simulink model "reachout_visual_rotation"  (Simulink 8.1)
settings: Solver=ode4  SolverMode=SingleTasking  StartTime=0.0  StopTime=inf  FixedStep=0.0005  RelTol=1e-3
model workspace (MAT data in the model file):
  BKIN_STEP_TIME = 0.0005
  col_x = 1
  col_y = 2
  E_TARGET_ON = 3
  E_HOLD_AT_TARGET = 5
  LOGICAL_RADIUS = 4
  START_TARGET_COL = 1
  END_TARGET_COL = 2
  ROTATION_CENTER = 3
  WAIT_AT_1stTARGET_COL = 4
  MAXREACHTIME_COL = 5
  WAIT_AT_2ndTARGET_COL = 6
  ROTATION_TYPE = 8
  ROTATION = 9
  DELAY_POSTTRIAL_COL = 7
  E_STAY_CENTER = 2
  VISUAL_RADIUS = 3
  COLOR = 5
  ALTCOLOR : num (value not decoded)
StartFcn:
  |  warndlg('Dexterit-E models cannot run under simulation. Please compile your model and run it from within Dexterit-E.');set_param(bdroot,'SimulationCommand','stop')
undefined symbols (not defined in the file or in its folder): slselsubs
libraries: General x3, Video x3, KINARM_general x1
CloseFcn:
  | rtwprivate ssgencode ModelCloseRequest b2lab2d
settings Model: Creator=Chris Grebeldinger  LastModifiedBy=dmclean  ModifiedComment=chris -- Wed Feb 16 09:18:30 2005 -- Version 1.1384  ModifiedHistory=Feb 16/05 - Add error repeat, add offset ramp  ExtModeArmWhenConnect=off  ExtModeLogAll=off  BufferReuse=off
settings DataIOCC: LimitDataPoints=off  SaveOutput=off  SaveTime=off  SignalLoggingName=sigsOut
settings OptimizationCC: BlockReduction=off  BooleanDataType=off  OptimizeBlockIOStorage=off  BufferReuse=off  ExpressionFolding=off  FoldNonRolledExpr=off  LocalBlockOutputs=off  InitFltsAndDblsToZero=on
settings DebuggingCC: SaveWithParameterizedLinksMsg=none  SignalResolutionControl=TryResolveAllWithWarning  SolverPrmCheckMsg=none  MultiTaskDSMMsg=warning  MultiTaskCondExecSysMsg=none  StrictBusMsg=None
settings HardwareCC: ProdIntDivRoundTo=Zero  ProdEndianess=LittleEndian  ProdHWDeviceType=Generic->32-bit x86 compatible  TargetHWDeviceType=32-bit Generic
settings SFSimCC: SimParseCustomCode=off
settings RTWCC: SystemTargetFile=xpctarget.tlc  TemplateMakefile=xpc_default_tmf  Description=xPC Target  ProcessScript=xpctarget_make_rtw_hook  IncludeERTFirstTime=on  RTWCompilerOptimization=On
settings CodeAppCC: MaxIdLength=63
settings xpcTargetCC: TargetFcnLib=ansi_tfl_tmw.mat  CodeReplacementLibrary=XPC_BLAS  ParMdlRefBuildCompliant=on  ConcurrentExecutionCompliant=on  CombineSignalStateStructs=off  MATLABClassNameForMDSCustomization=xpcAperiodicCustomization  GRTInterface=on  GenerateAllocFcn=off  xPCTaskExecutionProfile=off  xPCRL32EventNumber=5000  xPCisDownloadable=off  xPCLoadParamSetFile=off  xPCConcurrentTasks=off  xPCEnableSFAnimation=off

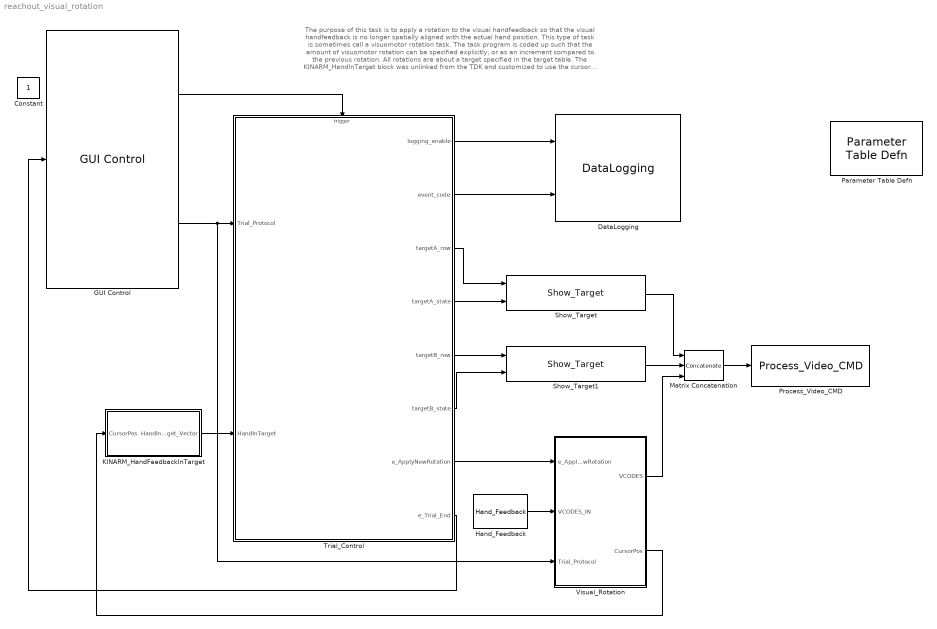
== system reachout_visual_rotation ==
  note: The purpose of this task is to apply a rotation to the visual handfeedback so that the visual handfeedback is no longer spatially aligned with the actual hand position.
      | This type of task is sometimes call a visuomotor rotation task.
      | The task program is coded up such that the amount of visuomotor rotation can be specified explicitly, or as an increment compared to the previous rotation.
      | All rotations are about a target specified in the target table.
      |
      | The KINARM_HandInTarget block was unlinked from the TDK and customized to use the cursor position as hand feedback input, rather than the KINARM robot's actual location.
  DataLogging : General/DataLogging  log_event_codes=on  log_analog_inputs=off
  GUI Control : General/GUI Control  target_type_str=Circle  Target_Type=1  XYcols=[1 2]  Vcols=3  Lcols=4  indices_padding=[0 0 0 0;0 0 0 0]  task_version=1.0  show_repeat_trial_flag=off
  Hand_Feedback : KINARM_general/Hand_Feedback  feedback_cntl_src=none
  KINARM_HandFeedbackInTarget : Subsystem  AncestorBlock=KINARM_general/KINARM_HandInTarget  mask(KINARM_HandInTarget){use_dominant_hand=on, target_type=Circle, num_states=1, attribcol1=4, attribcol2=3, attribcol3=3, attribcol4=3}
      mask prompts: use_dominant_hand "Dominant Hand?"; target_type "Type of Target"; num_states "Number of Target States"; attribcol1 "State 1 Target Table Column(s)"; attribcol2 "State 2 Target Table Column(s)"; attribcol3 "State 3 Target Table Column(s)"; attribcol4 "State 4 Target Table Column(s)"
      mask help: This block returns a vector or array corresponding to the Target_Table rows indicating whether the specified hand is in (=1) or out (=0) of each of the targets.
      mask init:
      | num_states=str2num(get_param(gcb, 'num_states'));
      | columntext='(columns: ';
      | 
      | for i=1:num_states
      | 	varname=['attribcol' num2str(i)];
      | 	if i>1
      | 		columntext=[columntext, '; '];
      | 	end
      | 	columntext=[columntext, get_param(gcb, varname)];
      | end
      | columntext=strvcat([columntext ')'],' ', ' ');
      | 
      | output_block=char(find_system(gcb,'LookUnderMasks','all','FollowLinks','on','SearchDepth',1,'BlockType','Outport'));
      | outputname=get_param(output_block,'Name');
      | 
      | % Select only the desired states for output. The output port is also renamed to reflect 
      | % whether the output is a vector (in the case of a single state) or an array (of vectors, 
      | % one for each of multiple states).
      | if num_states == 1
      | 	set_param([gcb '/Selected States'], 'Value', '[1]');
      | 	set_param(output_block, 'Name', 'HandInTarget_Vector');
      | elseif num_states == 2
      | 	set_param([gcb '/Selected States'], 'Value', '[1,2]');
      | 	set_param(output_block, 'Name', 'HandInTarget_Array');
      | elseif num_states == 3
      | 	set_param([gcb '/Selected States'], 'Value', '[1,2,3]');
      | 	set_param(output_block, 'Name', 'HandInTarget_Array');
      | else
      | 	set_param([gcb '/Selected States'], 'Value', '[1,2,3,4]');
      | 	set_param(output_block, 'Name', 'HandInTarget_Array');
      | end
      mask Help:
      | Used to determine if the hand (finger-tip) is in any of the targets in the Target_Table.
      | <P>
      | <B><I>Use of this block requires that the DataLogging block (General library) be set to log KINARM data.</I></B>
      | 
      | <H2>Library </H2>
      | KINARM_general (sub-library)
      | 
      | <H2>Description </H2>
      | This block returns a vector or array corresponding to the Target_Table rows indicating whether the specified hand (i.e. finger-tip) is in or out of each of the targets.  Each element in the output vector or output array will be either a 0 (hand not in target) or a 1 (hand in target).
      | <P>
      | A vector is returned if only one target state is specified in each target row (see Parameters and Dialog Box), with each index of the vector corresponding to a row in the target table.  An array is returned if more than one target state is specified in a target row, with each row of the array corresponding to a target row and each column corresponding to the nth target state specified in each target row.
      | <P>
      | The output vector or array is typically used by a stateflow chart to affect behavior of the system.  Because this block returns hand-in-target information for all targets in the target table, multiple targets can be monitored at once (i.e. the stateflow chart could have certain transitions that occur if the hand is in one target and other transitions if it is in a different target).  Likewise, because this block returns hand-in-target information for multiple states of a single target, those multiple states can be monitored simultaneously.
      | <P>
      | Because the KINARM_HandInTarget block returns information for only one hand, two copies of this block are required if information for both hands is desired.
      | <P>
      | 
      | <H2>Parameters and Dialog Box</H2>
      | <B>Dominant Hand?:</B> this box determines which hand is used by this block : dominant hand position (checked box) or the non-dominant hand position (unchecked box).  (Note: if the end-user wants to know about both the dominant hand and the non-dominant hand, then 2 separate copies of this block are requried, one for each hand.)
      | <P>
      | <B>Type of Target:</B> Enter the type of target specified in the target table:
      | <P>
      | <B>Number of Target States:</B> Enter the number of target states specified in each target row.  Up to four target states are allowed per target row.
      | <P>
      | <B>State <n> Target Table Columns:</B> Enter the columns in the Target Table that specify the relevant target attributes.  Do this for each target state.
      | For a circle, enter the columns corresponding to logical radius (e.g. 4)
      | <BR>For an ellipse, enter the columns corresponding to major radius, minor radius, rotation angle (e.g. [4, 5, 6]).
      | <BR>For a rectangle, enter the columns corresponding to length, height, and rotation angle (e.g. [4, 5, 6]).
      | <BR>For a line, enter the columns corresponding to stroke width, endpoint in x, and endpoint in y (e.g. [3, 4, 5]).
      | <BR>For a triangle, enter the columns corresponding to length, height, peak offset, and rotation angle (e.g. [4, 5, 6, 7]).
      | 
      | <H2>Examples</H2>
      | <B>Example 1.</B>  Suppose a target row will be used to define 1 state for a circle type target and the radius of the visual target is the same radius to be used for determination of hand-in-target.  The related Target Table column is: column 6 = radius.  For this example, "State 1 Target Table Columns" would equal [6].
      | <P>
      | 
      | <B>Example 2.</B>  Suppose a target row will be used to define 1 state for a circle type target, but the radius of the visual target will be different than the radius to be used for determination of hand-in-target.  This option allows independent control over the size of the visual target versus the accuracy needed to be considered "in the target".  The related Target Table columns are: column 6 = radius1 (i.e. radius to target to be drawn); column 7 = radius2 (i.e. radius to be used for hand-in-target) .  For this example, "State 1 Target Table Columns" would equal [7].
      | <P>
      | <B>Example 3.</B>  Suppose a target row will be used to define 2 states for a circle type target, where the radius of the visual target will be a constant, but depending on the state of the system, one of 2 other and different radii will be used for determination of hand-in-target.  The related Target Table columns are: column 6 = radius1 (i.e. radius to target to be drawn); column 7 = radius2 (i.e. radius to be used for hand-in-target for state 1); column 8 = radius3 (i.e. radius to be used for hand-in-target for state 2).  For this example, "State 1 Target Table Columns" would equal [7], while "State 2 Target Table Columns" would equal [8].
      | <P>
      | 
      | <H2>Related Blocks </H2>
      | DataLogging
      mask TypeOptions target_type: Circle | Ellipse | Rectangle | Line | Triangle
      mask Callback target_type:
      | target_type=get_param(gcb, 'target_type');
      | attribcol1=[str2num(get_param(gcb, 'attribcol1')) 0 0 0 0 0 0];
      | attribcol2=[str2num(get_param(gcb, 'attribcol2')) 0 0 0 0 0 0];
      | attribcol3=[str2num(get_param(gcb, 'attribcol3')) 0 0 0 0 0 0];
      | attribcol4=[str2num(get_param(gcb, 'attribcol4')) 0 0 0 0 0 0];
      | switch target_type(1:3)
      | 	case 'Cir'
      | 		numcol=1;
      | 	case 'Ell'
      | 		numcol=3;
      |     case 'Rec'
      |         numcol=3;
      |     case 'Lin'
      |         numcol=3;
      |     case 'Tri'
      |         numcol=4;
      | 	otherwise
      | 		numcol=1;
      | end
      | if numcol==1
      | 	set_param(gcb, 'attribcol1', num2str(attribcol1(1)));
      | 	set_param(gcb, 'attribcol2', num2str(attribcol2(1)));
      | 	set_param(gcb, 'attribcol3', num2str(attribcol3(1)));
      | 	set_param(gcb, 'attribcol4', num2str(attribcol4(1)));
      | else
      | 	set_param(gcb, 'attribcol1', ['[' num2str(attribcol1(1:numcol)) ']']);
      | 	set_param(gcb, 'attribcol2', ['[' num2str(attribcol2(1:numcol)) ']']);
      | 	set_param(gcb, 'attribcol3', ['[' num2str(attribcol3(1:numcol)) ']']);
      | 	set_param(gcb, 'attribcol4', ['[' num2str(attribcol4(1:numcol)) ']']);
      | end
      mask TypeOptions num_states: 1 | 2 | 3 | 4
      mask Callback num_states:
      | num_states = str2num(get_param(gcb, 'num_states'));
      | vis = get_param(gcb, 'MaskVisibilities');
      | 
      | % Select only the desired states for output. The output port is also renamed to reflect
      | % whether the output is a vector (in the case of a single state) or an array (of vectors,
      | % one for each of multiple states).
      | output_block=char(find_system(gcb, 'LookUnderMasks', 'all', 'FollowLinks', 'on', 'SearchDepth', 1, 'BlockType', 'Outport'));
      | 
      | if num_states == 1
      | 	set_param([gcb '/Selected States'], 'Value', '[1]');
      | 	set_param(output_block, 'Name', 'HandInTarget_Vector');
      | 	vis{5} = 'off';
      | 	vis{6} = 'off';
      | 	vis{7} = 'off';
      | elseif num_states == 2
      | 	set_param([gcb '/Selected States'], 'Value', '[1,2]');
      | 	set_param(output_block, 'Name', 'HandInTarget_Array');
      | 	vis{5} = 'on';
      | 	vis{6} = 'off';
      | 	vis{7} = 'off';
      | elseif num_states == 3
      | 	set_param([gcb '/Selected States'], 'Value', '[1,2,3]');
      | 	set_param(output_block, 'Name','HandInTarget_Array');
      | 	vis{5} = 'on';
      | 	vis{6} = 'on';
      | 	vis{7} = 'off';
      | else
      | 	set_param([gcb '/Selected States'], 'Value', '[1,2,3,4]');
      | 	set_param(output_block, 'Name', 'HandInTarget_Array');
      | 	vis{5} = 'on';
      | 	vis{6} = 'on';
      | 	vis{7} = 'on';
      | end
      | set_param(gcb, 'MaskVisibilities', vis);
      | 
      | target_type=get_param(gcb, 'target_type');
      | attribcol1=[str2num(get_param(gcb, 'attribcol1')) 0 0 0 0 0 0];
      | attribcol2=[str2num(get_param(gcb, 'attribcol2')) 0 0 0 0 0 0];
      | attribcol3=[str2num(get_param(gcb, 'attribcol3')) 0 0 0 0 0 0];
      | attribcol4=[str2num(get_param(gcb, 'attribcol4')) 0 0 0 0 0 0];
      | switch target_type(1:3)
      | 	case 'Cir'
      | 		numcol=1;
      | 	case 'Ell'
      | 		numcol=3;
      |     case 'Rec'
      |         numcol=3;
      |     case 'Lin'
      |         numcol=3;
      |     case 'Tri'
      |         numcol=4;
      | 	otherwise
      | 		numcol=1;
      | end
      | if numcol==1
      | 	set_param(gcb, 'attribcol1', num2str(attribcol1(1)));
      | 	set_param(gcb, 'attribcol2', num2str(attribcol2(1)));
      | 	set_param(gcb, 'attribcol3', num2str(attribcol3(1)));
      | 	set_param(gcb, 'attribcol4', num2str(attribcol4(1)));
      | else
      | 	set_param(gcb, 'attribcol1', ['[' num2str(attribcol1(1:numcol)) ']']);
      | 	set_param(gcb, 'attribcol2', ['[' num2str(attribcol2(1:numcol)) ']']);
      | 	set_param(gcb, 'attribcol3', ['[' num2str(attribcol3(1:numcol)) ']']);
      | 	set_param(gcb, 'attribcol4', ['[' num2str(attribcol4(1:numcol)) ']']);
      | end
      mask Callback attribcol1:
      | target_type=get_param(gcb, 'target_type');
      | attribcol1=[str2num(get_param(gcb, 'attribcol1')) 0 0 0 0 0 0];
      | attribcol2=[str2num(get_param(gcb, 'attribcol2')) 0 0 0 0 0 0];
      | attribcol3=[str2num(get_param(gcb, 'attribcol3')) 0 0 0 0 0 0];
      | attribcol4=[str2num(get_param(gcb, 'attribcol4')) 0 0 0 0 0 0];
      | switch target_type(1:3)
      | 	case 'Cir'
      | 		numcol=1;
      | 	case 'Ell'
      | 		numcol=3;
      |     case 'Rec'
      |         numcol=3;
      |     case 'Lin'
      |         numcol=3;
      |     case 'Tri'
      |         numcol=4;
      | 	otherwise
      | 		numcol=1;
      | end
      | if numcol==1
      | 	set_param(gcb, 'attribcol1', num2str(attribcol1(1)));
      | 	set_param(gcb, 'attribcol2', num2str(attribcol2(1)));
      | 	set_param(gcb, 'attribcol3', num2str(attribcol3(1)));
      | 	set_param(gcb, 'attribcol4', num2str(attribcol4(1)));
      | else
      | 	set_param(gcb, 'attribcol1', ['[' num2str(attribcol1(1:numcol)) ']']);
      | 	set_param(gcb, 'attribcol2', ['[' num2str(attribcol2(1:numcol)) ']']);
      | 	set_param(gcb, 'attribcol3', ['[' num2str(attribcol3(1:numcol)) ']']);
      | 	set_param(gcb, 'attribcol4', ['[' num2str(attribcol4(1:numcol)) ']']);
      | end
      mask Callback attribcol2:
      | target_type=get_param(gcb, 'target_type');
      | attribcol1=[str2num(get_param(gcb, 'attribcol1')) 0 0 0 0 0 0];
      | attribcol2=[str2num(get_param(gcb, 'attribcol2')) 0 0 0 0 0 0];
      | attribcol3=[str2num(get_param(gcb, 'attribcol3')) 0 0 0 0 0 0];
      | attribcol4=[str2num(get_param(gcb, 'attribcol4')) 0 0 0 0 0 0];
      | switch target_type(1:3)
      | 	case 'Cir'
      | 		numcol=1;
      | 	case 'Ell'
      | 		numcol=3;
      |     case 'Rec'
      |         numcol=3;
      |     case 'Lin'
      |         numcol=3;
      |     case 'Tri'
      |         numcol=4;
      | 	otherwise
      | 		numcol=1;
      | end
      | if numcol==1
      | 	set_param(gcb, 'attribcol1', num2str(attribcol1(1)));
      | 	set_param(gcb, 'attribcol2', num2str(attribcol2(1)));
      | 	set_param(gcb, 'attribcol3', num2str(attribcol3(1)));
      | 	set_param(gcb, 'attribcol4', num2str(attribcol4(1)));
      | else
      | 	set_param(gcb, 'attribcol1', ['[' num2str(attribcol1(1:numcol)) ']']);
      | 	set_param(gcb, 'attribcol2', ['[' num2str(attribcol2(1:numcol)) ']']);
      | 	set_param(gcb, 'attribcol3', ['[' num2str(attribcol3(1:numcol)) ']']);
      | 	set_param(gcb, 'attribcol4', ['[' num2str(attribcol4(1:numcol)) ']']);
      | end
      mask Callback attribcol3:
      | target_type=get_param(gcb, 'target_type');
      | attribcol1=[str2num(get_param(gcb, 'attribcol1')) 0 0 0 0 0 0];
      | attribcol2=[str2num(get_param(gcb, 'attribcol2')) 0 0 0 0 0 0];
      | attribcol3=[str2num(get_param(gcb, 'attribcol3')) 0 0 0 0 0 0];
      | attribcol4=[str2num(get_param(gcb, 'attribcol4')) 0 0 0 0 0 0];
      | switch target_type(1:3)
      | 	case 'Cir'
      | 		numcol=1;
      | 	case 'Ell'
      | 		numcol=3;
      |     case 'Rec'
      |         numcol=3;
      |     case 'Lin'
      |         numcol=3;
      |     case 'Tri'
      |         numcol=4;
      | 	otherwise
      | 		numcol=1;
      | end
      | if numcol==1
      | 	set_param(gcb, 'attribcol1', num2str(attribcol1(1)));
      | 	set_param(gcb, 'attribcol2', num2str(attribcol2(1)));
      | 	set_param(gcb, 'attribcol3', num2str(attribcol3(1)));
      | 	set_param(gcb, 'attribcol4', num2str(attribcol4(1)));
      | else
      | 	set_param(gcb, 'attribcol1', ['[' num2str(attribcol1(1:numcol)) ']']);
      | 	set_param(gcb, 'attribcol2', ['[' num2str(attribcol2(1:numcol)) ']']);
      | 	set_param(gcb, 'attribcol3', ['[' num2str(attribcol3(1:numcol)) ']']);
      | 	set_param(gcb, 'attribcol4', ['[' num2str(attribcol4(1:numcol)) ']']);
      | end
      mask Callback attribcol4:
      | target_type=get_param(gcb, 'target_type');
      | attribcol1=[str2num(get_param(gcb, 'attribcol1')) 0 0 0 0 0 0];
      | attribcol2=[str2num(get_param(gcb, 'attribcol2')) 0 0 0 0 0 0];
      | attribcol3=[str2num(get_param(gcb, 'attribcol3')) 0 0 0 0 0 0];
      | attribcol4=[str2num(get_param(gcb, 'attribcol4')) 0 0 0 0 0 0];
      | switch target_type(1:3)
      | 	case 'Cir'
      | 		numcol=1;
      | 	case 'Ell'
      | 		numcol=3;
      |     case 'Rec'
      |         numcol=3;
      |     case 'Lin'
      |         numcol=3;
      |     case 'Tri'
      |         numcol=4;
      | 	otherwise
      | 		numcol=1;
      | end
      | if numcol==1
      | 	set_param(gcb, 'attribcol1', num2str(attribcol1(1)));
      | 	set_param(gcb, 'attribcol2', num2str(attribcol2(1)));
      | 	set_param(gcb, 'attribcol3', num2str(attribcol3(1)));
      | 	set_param(gcb, 'attribcol4', num2str(attribcol4(1)));
      | else
      | 	set_param(gcb, 'attribcol1', ['[' num2str(attribcol1(1:numcol)) ']']);
      | 	set_param(gcb, 'attribcol2', ['[' num2str(attribcol2(1:numcol)) ']']);
      | 	set_param(gcb, 'attribcol3', ['[' num2str(attribcol3(1:numcol)) ']']);
      | 	set_param(gcb, 'attribcol4', ['[' num2str(attribcol4(1:numcol)) ']']);
      | end
      mask Display:
      | disp(columntext)
      | port_label('output',1,outputname)
  Matrix Concatenation : Concatenate  NumInputs=3  Mode=Multidimensional array
  Parameter Table Defn : General/Parameter Table Defn  ShowInLibBrowser=0
  Process_Video_CMD : Video/Process_Video_CMD
  Show_Target : Video/Show_Target  target_type=Circle  num_states=2  attribcol1=[COLOR 0 0 VISUAL_RADIUS]  attribcol2=[ALTCOLOR 0 0 VISUAL_RADIUS]  attribcol3=[0 0 0 0]  attribcol4=[0 0 0 0]  attribcol5=[0 0 24 0]  stateindices_padding=[0 0 0 0 0 0 0;0 0 0 0 0 0 0;0 0 0 0 0 0 0;0 0 0 0 0 0 0;0 0 0 0 0 0 0]  source=dialog  opacity=100  target_display=Both subject and operator displays  num_col=4
  Show_Target1 : Video/Show_Target  target_type=Circle  num_states=2  attribcol1=[COLOR 0 0 VISUAL_RADIUS]  attribcol2=[ALTCOLOR 0 0 VISUAL_RADIUS]  attribcol3=[0 0 0 0]  attribcol4=[0 0 0 0]  attribcol5=[0 0 24 0]  stateindices_padding=[0 0 0 0 0 0 0;0 0 0 0 0 0 0;0 0 0 0 0 0 0;0 0 0 0 0 0 0;0 0 0 0 0 0 0]  source=dialog  opacity=100  target_display=Both subject and operator displays  num_col=4
  Trial_Control : Stateflow chart  TreatAsAtomicUnit=on
  Visual_Rotation : Subsystem
  Constant : Constant  IOType=siggen
  wires:
  Show_Target/1 -> Matrix Concatenation/1
  GUI Control/2 -> Trial_Control/1(Trial_Protocol), Visual_Rotation/3(Trial_Protocol)
  Trial_Control/8(e_Trial_End) -> GUI Control/1
  GUI Control/1 -> Trial_Control/Trigger
  Trial_Control/4(targetA_state) -> Show_Target/2
  Trial_Control/3(targetA_row) -> Show_Target/1
  Show_Target1/1 -> Matrix Concatenation/2
  Trial_Control/5(targetB_row) -> Show_Target1/1
  Trial_Control/6(targetB_state) -> Show_Target1/2
  Trial_Control/2(event_code) -> DataLogging/2
  Matrix Concatenation/1 -> Process_Video_CMD/1
  Hand_Feedback/1 -> Visual_Rotation/2(VCODES_IN)
  Visual_Rotation/2(CursorPos) -> KINARM_HandFeedbackInTarget/1(CursorPos)
  KINARM_HandFeedbackInTarget/1(HandInTarget_Vector) -> Trial_Control/2(HandInTarget)
  Trial_Control/7(e_ApplyNewRotation) -> Visual_Rotation/1(e_ApplyNewRotation)
  Visual_Rotation/1(VCODES) -> Matrix Concatenation/3
  Trial_Control/1(logging_enable) -> DataLogging/1

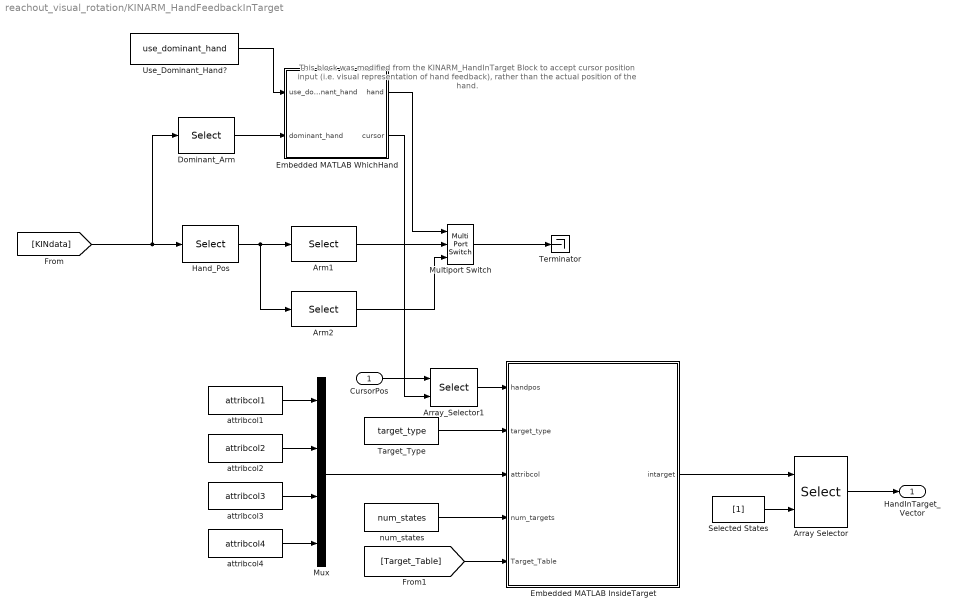
== system reachout_visual_rotation/KINARM_HandFeedbackInTarget ==
  note: This block was modified from the KINARM_HandInTarget Block to accept cursor position input (i.e. visual
      | representation of hand feedback), rather than the actual position of the hand.
  CursorPos : Inport
  Arm1 : Selector  NumberOfDimensions=2  InputPortWidth=3  IndexOptions=Index vector (dialog),Select all  Indices=1,-1  OutputSizes=slselsubs([(-2),(-2)],1),slselsubs([(-2),(-2)],2)
  Arm2 : Selector  NumberOfDimensions=2  InputPortWidth=3  IndexOptions=Index vector (dialog),Select all  Indices=2,-1  OutputSizes=slselsubs([(-2),(-2)],1),slselsubs([(-2),(-2)],2)
  Array Selector : Selector  NumberOfDimensions=2  InputPortWidth=3  IndexOptions=Select all,Index vector (port)  Indices=-1,1  OutputSizes=slselsubs([(-2),(-2)],1),slselsubs([(-2),(-2)],2)
  Array_Selector1 : Selector  NumberOfDimensions=2  InputPortWidth=3  IndexOptions=Index vector (port),Select all  Indices=-1,1  OutputSizes=1
  Dominant_Arm : Selector  NumberOfDimensions=2  InputPortWidth=3  IndexOptions=Index vector (dialog),Index vector (dialog)  Indices=[3],[1]  OutputSizes=slselsubs([(-2),(-2)],1),slselsubs([(-2),(-2)],2)
  Embedded MATLAB InsideTarget : MATLAB Function  TreatAsAtomicUnit=on
  Embedded MATLAB WhichHand : MATLAB Function  TreatAsAtomicUnit=on
  Hand_Pos : Selector  NumberOfDimensions=2  InputPortWidth=3  IndexOptions=Select all,Index vector (dialog)  Indices=-1,[23,24]  OutputSizes=slselsubs([(-2),(-2)],1),slselsubs([(-2),(-2)],2)
  Multiport Switch : MultiPortSwitch  Inputs=2
  Mux : Mux
  Selected States : Constant  Value=[1]
  Target_Type : Constant  Value=target_type
  Terminator : Terminator
  Use_Dominant_Hand? : Constant  Value=use_dominant_hand
  attribcol1 : Constant  Value=attribcol1
  attribcol2 : Constant  Value=attribcol2
  attribcol3 : Constant  Value=attribcol3
  attribcol4 : Constant  Value=attribcol4
  num_states : Constant  Value=num_states
  HandInTarget_Vector : Outport
  wires:
  Selected States/1 -> Array Selector/2
  num_states/1 -> Embedded MATLAB InsideTarget/4(num_targets)
  Mux/1 -> Embedded MATLAB InsideTarget/3(attribcol)
  attribcol4/1 -> Mux/4
  attribcol3/1 -> Mux/3
  attribcol2/1 -> Mux/2
  attribcol1/1 -> Mux/1
  Use_Dominant_Hand?/1 -> Embedded MATLAB WhichHand/1(use_dominant_hand)
  Embedded MATLAB WhichHand/1(hand) -> Multiport Switch/1
  Target_Type/1 -> Embedded MATLAB InsideTarget/2(target_type)
  Array Selector/1 -> HandInTarget_Vector/1
  [Target_Table] -> Embedded MATLAB InsideTarget/5(Target_Table)
  Embedded MATLAB InsideTarget/1(intarget) -> Array Selector/1
  Multiport Switch/1 -> Terminator/1
  Arm2/1 -> Multiport Switch/3
  Arm1/1 -> Multiport Switch/2
  Dominant_Arm/1 -> Embedded MATLAB WhichHand/2(dominant_hand)
  Hand_Pos/1 -> Arm2/1, Arm1/1
  [KINdata] -> Dominant_Arm/1, Hand_Pos/1
  CursorPos/1 -> Array_Selector1/1
  Array_Selector1/1 -> Embedded MATLAB InsideTarget/1(handpos)
  Embedded MATLAB WhichHand/2(cursor) -> Array_Selector1/2

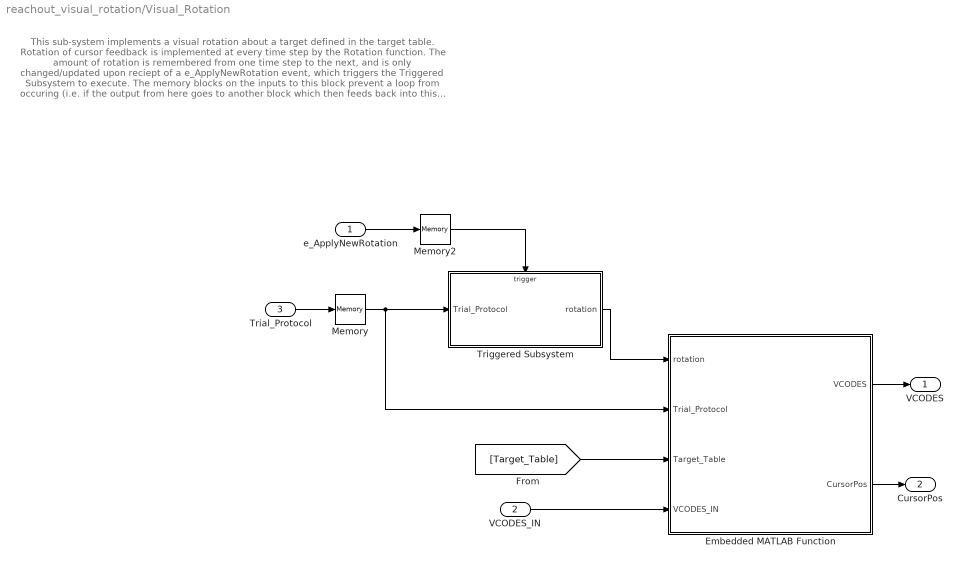
== system reachout_visual_rotation/Visual_Rotation ==
  note: This sub-system implements a visual rotation about a target defined in the target table.
      |
      | Rotation of cursor feedback is implemented at every time step by the Rotation function.
      | The amount of rotation is remembered from one time step to the next, and is only changed/updated
      | upon reciept of a e_ApplyNewRotation event, which triggers the Triggered Subsystem to execute.
      |
      | The memory blocks on the inputs to this block prevent a loop from occuring (i.e. if the output from here goes to
      | another block which then feeds back into this block, which forms a loop, which needs to be broken by the Memory block).
  e_ApplyNewRotation : Inport
  VCODES_IN : Inport  Port=2
  Trial_Protocol : Inport  Port=3
  Embedded MATLAB Function : MATLAB Function  TreatAsAtomicUnit=on
  Memory : Memory  InheritSampleTime=on
  Memory2 : Memory  InheritSampleTime=on
  Triggered Subsystem : Subsystem  TreatAsAtomicUnit=on
  VCODES : Outport
  CursorPos : Outport  Port=2
  wires:
  Trial_Protocol/1 -> Memory/1
  Embedded MATLAB Function/1(VCODES) -> VCODES/1
  VCODES_IN/1 -> Embedded MATLAB Function/4(VCODES_IN)
  Embedded MATLAB Function/2(CursorPos) -> CursorPos/1
  Memory/1 -> Triggered Subsystem/1(Trial_Protocol), Embedded MATLAB Function/2(Trial_Protocol)
  e_ApplyNewRotation/1 -> Memory2/1
  Triggered Subsystem/1(rotation) -> Embedded MATLAB Function/1(rotation)
  [Target_Table] -> Embedded MATLAB Function/3(Target_Table)
  Memory2/1 -> Triggered Subsystem/Trigger

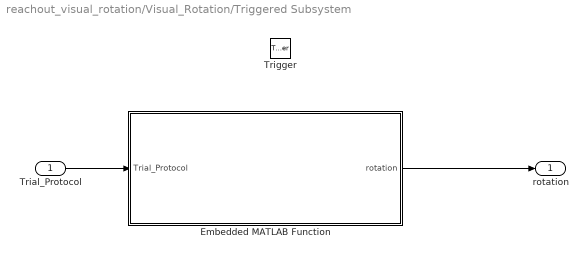
== system reachout_visual_rotation/Visual_Rotation/Triggered Subsystem ==
  Trial_Protocol : Inport
  Trigger : TriggerPort  TriggerType=either
  Embedded MATLAB Function : MATLAB Function  TreatAsAtomicUnit=on
  rotation : Outport
  wires:
  Trial_Protocol/1 -> Embedded MATLAB Function/1(Trial_Protocol)
  Embedded MATLAB Function/1(rotation) -> rotation/1

== stateflow chart Trial_Control ==
  settings: sampleTime=0.001
  state Inter_Trial_State/
    // send e_Trial_End event
    e_Trial_End;
    // turn off both targets
    // stop data logging
    event_code=0;
    targetA_state=0;
    targetB_state=0;
    logging_enable = 0;
  state Initialize/
    // Turn off both targets, set hand_feedback on
    targetA_state=0;
    targetB_state=0;
  state Main_Trial
    state Show2ndTarget/
      // Turn on second target, log an event, wait until hand-is-in-target or wait for specified delay
      event_code=E_TARGET_ON;
      targetB_row = Trial_Protocol[END_TARGET_COL];
      targetB_state=1;
      tickCount =Trial_Protocol[MAXREACHTIME_COL];
    state StayAt2ndTarget/
      // change the 2nd target's state, log an event, wait for a specified period of time
      event_code=E_HOLD_AT_TARGET;
      targetB_state=2;
      tickCount =Trial_Protocol[WAIT_AT_2ndTARGET_COL];
    state EndOfTrial/
      // Wait for a specified period of time,
      tickCount =Trial_Protocol[DELAY_POSTTRIAL_COL];
    state StayAtFirstTarget/
      // change the first target state (e.g. colour), log an event, wait for specified period of time.  Hand must STAY in target for specified time.
      logging_enable = 1;
      event_code=E_STAY_CENTER;
      targetA_state=2;
      tickCount =Trial_Protocol[WAIT_AT_1stTARGET_COL];
    state FirstTargetOn/
      // Turn on first target, set loading conditions, enable data logging, wait for specified delay or until hand-is-in-target
      targetA_row = Trial_Protocol[START_TARGET_COL];
      targetA_state=1;
    FirstTargetOn -> StayAtFirstTarget : [HandInTarget[targetA_row]==1]
    StayAtFirstTarget -> FirstTargetOn [order 2] : [HandInTarget[targetA_row]==0]
    StayAtFirstTarget -> Show2ndTarget [order 1] : after(tickCount, e_clk)/
        | e_ApplyNewRotation
        | // apply the new rotation amount now (i.e. wait until the subject is in the starting target before applying a new
        | // rotation, so that they do not see the hand feedback jump/change when a new rotation is applied)
        | // have this event occur on this transition, rather than in the "StayAtFirstTarget" state to ensure that the subject
        | // is really starting the trial.  Could have put this event in the "Show2ndTarget" state instead.
    Show2ndTarget -> StayAt2ndTarget [order 2] : [HandInTarget[targetB_row]==1]
    Show2ndTarget -> EndOfTrial [order 1] : after(tickCount, e_clk)/
    StayAt2ndTarget -> EndOfTrial : after(tickCount, e_clk)
  (default) -> Initialize
  Initialize -> FirstTargetOn
  Inter_Trial_State -> FirstTargetOn : after(tickCount, e_clk)
  Main_Trial -> Inter_Trial_State : e_ExitTrialNow/
      | // if e_ExitTrialNow event occurs...
      | tickCount=1;
  EndOfTrial -> Inter_Trial_State
  data: logging_enable output boolean; event_code output uint16 [0..] =0; Trial_Protocol input double; HandInTarget input double; targetA_row output double [1..32]; targetA_state output double; targetB_row output double; targetB_state output double; tickCount local double
  data targetA_row settings: description=index of the row currently being used in the TargetTable
  events: e_ApplyNewRotation output EITHER_EDGE_EVENT; e_clk input RISING_EDGE_EVENT; e_ExitTrialNow input EITHER_EDGE_EVENT; e_Trial_End output EITHER_EDGE_EVENT

== matlab function Visual_Rotation/Triggered Subsystem/Embedded MATLAB Function ==
  settings: fimath=|
      | fimath(...
      | 'RoundMode', 'floor',...
      | 'OverflowMode', 'wrap',...
      | 'ProductMode', 'KeepLSB', 'ProductWordLength', 32,...
      | 'SumMode', 'KeepLSB', 'SumWordLength', 32,...
      | 'CastBeforeSum', false)
  data: rotation output double; Trial_Protocol input double
function rotation   = Calculate_Desired_Rotation(Trial_Protocol)
% This block supports an embeddable subset of the MATLAB language.
% See the help menu for details. 

%This block was modified by IEB, Sept 24, 2008
%It updates the desired amount of rotation

% NOTE ALL ROTATIONS ARE CURRENTLY IN DEGREES IN THE FUNCTION

% create a persistent variable to remember the rotation amount from one time-step to the next
persistent rotation_memory

if isempty(rotation_memory),            rotation_memory = 0;										end

% where to look in the TP table for these parameters
rotate_type_COL = 8;
rotation_amount_COL = 9;

rotate_type = Trial_Protocol(rotate_type_COL);
rotation_amount = Trial_Protocol(rotation_amount_COL);

if rotate_type == 0
	%set the rotation = 0
	rotation = 0;
elseif rotate_type ==1
	%set the rotation = specified amount
	rotation = rotation_amount;
elseif rotate_type == 2
	%set the rotation to change by specified amount
	rotation = rotation_memory + rotation_amount;
else
	%do nothing
	rotation = rotation_memory;
end

% save the rotation amount for the next time-step
rotation_memory = rotation;

== matlab function Visual_Rotation/Embedded MATLAB Function ==
  settings: fimath=|
      | fimath(...
      | 'RoundMode', 'floor',...
      | 'OverflowMode', 'wrap',...
      | 'ProductMode', 'KeepLSB', 'ProductWordLength', 32,...
      | 'SumMode', 'KeepLSB', 'SumWordLength', 32,...
      | 'CastBeforeSum', false)
  data: VCODES output double; rotation input double; Trial_Protocol input double; Target_Table input double; CursorPos output double; VCODES_IN input double
function [VCODES, CursorPos]  = Rotation(rotation, Trial_Protocol, Target_Table, VCODES_IN)
% This block supports an embeddable subset of the MATLAB language.
% See the help menu for details. 

%This block was modified by IEB, Sept 24, 2008
%It rotates the cursor position around a location specified as a target in the Trial_Protocol.

% VCODEs are length VCODE_LENGTH.
% All dimensions are units of (m).
% VCODE index definition: 1-5 as the same for all target types
% 1 - Target type
%		1=circle
%		2=ellipse
%       3=rectangle
%		4=line
%       5=triangle
%		6 and higher - not implemented yet
% 2 - status
%		0=off
%		1=on
% 3 - x position (m)
% 4 - y position (m)

% column in target table to find the target to rotation about
rotation_center_COL = 3;

rotation_center_target = Trial_Protocol(rotation_center_COL);
x_center = Target_Table(rotation_center_target, 1) * 0.01;		%convert to meters
y_center = Target_Table(rotation_center_target, 2) * 0.01;		%convert to meters

rotation = rotation*pi/180;		%convert desired rotation from degrees to radians

VCODES = VCODES_IN;
CursorPos = VCODES(1:2,3:4);
T = [x_center, y_center; x_center, y_center];                       %translation matrix
R = [cos(rotation) -sin(rotation); sin(rotation) cos(rotation)];	%rotation matrix

CursorPos = CursorPos - T;				%translate
CursorPos = (R*CursorPos')';			%rotate
CursorPos = CursorPos + T;				%re-translate

VCODES(1:2,3:4) = CursorPos;			%apply updated positions back into the VCODEs

== matlab function KINARM_HandFeedbackInTarget/Embedded MATLAB InsideTarget ==
  settings: fimath=|
      | fimath(...
      | 'RoundMode', 'floor',...
      | 'OverflowMode', 'wrap',...
      | 'ProductMode', 'KeepLSB', 'ProductWordLength', 32,...
      | 'SumMode', 'KeepLSB', 'SumWordLength', 32,...
      | 'CastBeforeSum', false)
  data: handpos input double size=2; target_type input double; attribcol input double; num_targets input double; intarget output double; Target_Table input double
function intarget = FIsInsideTarget(handpos, target_type, attribcol, num_targets, Target_Table)
% all dimensions in m, rad
% arguments:
% handpos: x,y positions of center of target
% attribcol: columns in target table specifying target attributes.  
% Specific to Target_Type
%	circle:
%	[X0,Y0,r...,rn] where:
%	X0,Y0 : centre of circle
%	r : logical radius of circle (i.e. radius used to determine 'in' or 'out' of target)
%	rn: logical radius of other targets (e.g. 2nd, 3rd) also specified in target row.
%   Up to 4 targets can be specified in a row
% ellipse:
%	[X0,Y0,a,b,t...,an, bn, tn] where:
%	X0,Y0 : centre of ellipse
%	a,b : major, minor radii of ellipse
%	t : rotation of ellipse in degrees
%	an,bn : major, minor radii of ellipse of other targets (e.g. 2nd, 3rd) also specified in target row
%	tn : rotation of ellipse in degrees of other targets (e.g. 2nd, 3rd) also specified in target row
%   Up to 4 targets can be specified in a row


target_col_x=1;
target_col_y=2;

x=handpos(1);
y=handpos(2);

intarget = zeros(size(Target_Table,1),4);

X0 = Target_Table(:,target_col_x)*0.01;			%Target Table sizes in cm in v1.4
Y0 = Target_Table(:,target_col_y)*0.01;			%Target Table sizes in cm in v1.4

deltax=x-X0;
deltay=y-Y0;

INT_MAX=2^32-1;

if target_type==1			%circle
	for target=1:num_targets
		r = Target_Table(:,attribcol(target))*0.01;			%Target Table sizes in cm in v1.4
		% simple euclidean distance
		distance2 = deltax.^2 + deltay.^2;					%distance2 is the square of the distance
	    intarget(:,target) = (distance2 <= r.^2);
	end
elseif target_type==2		%ellipse
	for target=1:num_targets
	    a = Target_Table(:,attribcol(target*3-2))*0.01;			%Target Table sizes in cm in v1.4
	    b = Target_Table(:,attribcol(target*3-1))*0.01;			%Target Table sizes in cm in v1.4	
	    t = Target_Table(:,attribcol(target*3))*(pi / 180.0);	%Target Table angles in degrees in v1.4
		sint=sin(t);
		cost=cos(t);
		xrotate=deltax.*cost+deltay.*sint;		%location of x point in ellipse's coordinate frame
		yrotate=-deltax.*sint+deltay.*cost;		%location of y point in ellipse's coordinate frame
		m=yrotate./xrotate;						%slope of line between the (x,y) to (x0,y0) in ellipse's coordinate frame
		y2sq=1./(1./(m.*a).^2+1./b.^2);			%y2sq is y2^2, where y2 is the intersection of the ellipse and the (x,y) to (x0,y0) line
	    intarget(:,target) = (yrotate.^2 <= y2sq);
    end
elseif target_type==3       %rectangle
    for target=1:num_targets
        w = Target_Table(:,attribcol(target*3-2))*0.01;  %width (sizes in cm in v1.4)
        h = Target_Table(:,attribcol(target*3-1))*0.01;  %height (sizes in cm in v1.4)
        
        if attribcol(target*3) > 0
            t = Target_Table(:,attribcol(target*3))*(pi / 180.0);  %angle (angles in degrees in v1.4)
        else
            t = zeros(size(Target_Table, 1), 1);
        end

        sint=sin(t);
        cost=cos(t);

        xrotate=deltax.*cost + deltay.*sint;   %location of x point in rectangle's coordinate frame
        yrotate=-deltax.*sint + deltay.*cost;  %location of y point in rectangle's coordinate frame

        intarget(:,target) = abs(xrotate) <= w/2 & abs(yrotate) <= h/2;
    end
elseif target_type==4       %line
    for target=1:num_targets
        % treat the line like a rectangle of height h and width w
        % determine height (stroke width) in the same fashion as in Show_Target
        if attribcol(target*3-2) == 0                     %0 column index means stroke width of 0
            h = zeros(size(Target_Table, 1), 1);
        elseif attribcol(target*3-2) < 0                  %-ve column index means stroke width of 1mm
            h = ones(size(Target_Table, 1), 1) .* 0.001;
        else
            h = Target_Table(:,attribcol(target*3-2)) * 0.01;  %target table contains width in cm
        end
        
        ex = Target_Table(:,attribcol(target*3-1))*0.01;  %endpoint in x relative to start point (cm)
        ey = Target_Table(:,attribcol(target*3))*0.01;    %endpoint in y relative to start point (cm)
        
        w = sqrt(ex.^2 + ey.^2);                          %width (cm)
        
        % determine the vector from the line's midpoint to the hand position
        handx = deltax - ex/2;
        handy = deltay - ey/2;
        
        t = atan2(ey, ex);                                %calculate angle of the line (rads)
        sint = sin(t);
        cost = cos(t);
        
        xrotate = handx.*cost + handy.*sint;   %location of x point in rectangle's coordinate frame
        yrotate = -handx.*sint + handy.*cost;  %location of y point in rectangle's coordinate frame
 
        intarget(:,target) = abs(xrotate) <= w/2 & abs(yrotate) <= h/2;
    end
elseif target_type==5  % triangle
    for target=1:num_targets
        w = Target_Table(:,attribcol(target*4-3))*0.01;         %length (sizes in cm in v1.4)
        
        % If a height column of 0 is specified, make the triangle equilateral. Otherwise, use the
        % values for height and peak offset from the target table.
        if attribcol(target*4-2) > 0
            h = Target_Table(:,attribcol(target*4-2))*0.01;  %height (sizes in cm in v1.4)
            p = Target_Table(:,attribcol(target*4-1))*0.01;  %peak offset (sizes in cm in v1.4)
        else
            h = w.*sin(pi/3.0);
            p = zeros(size(Target_Table, 1), 1);
        end
        
        if attribcol(target*4) > 0
            t = Target_Table(:,attribcol(target*4))*(pi / 180.0);  %angle (angles in degrees in v1.4)
        else
            t = zeros(size(Target_Table, 1), 1);
        end
        
        sint = sin(t);
        cost = cos(t);
        
        xrotate = deltax.*cost + deltay.*sint;   %location of x point in triangle's coordinate frame
        yrotate = -deltax.*sint + deltay.*cost;  %location of y point in triangle's coordinate frame
        
        % Begin to find centroid of triangle relative to the point on the base beneath the peak. "Left vertex" 
        % refers to the vertex at the left end of the base, and "right vertex" to the vertex at the right end.
        n = w./2.0 + p;  % distance along base from left vertex to peak
        m = w./2.0 - p;  % distance along base from peak to right vertex

        alpha = atan2(h, n);  % angle between base and line from left vertex to peak
        beta = atan2(h, m);   % angle between base and line from right vertex to peak
        
        length1 = sqrt(h.*h + n.*n) ./ 2.0;  % half length of line from left vertex to peak
        length2 = sqrt(h.*h + m.*m) ./ 2.0;  % half length of line from right vertex to peak

        % Determine slope of line from left vertex to midpoint of line from right vertex to peak.
        slope1 = ones(size(Target_Table, 1), 1) .* INT_MAX;
        
        for i=1:size(Target_Table, 1)
            if abs(w(i) - length2(i)*cos(beta(i))) > 0.0
                slope1(i) = length2(i)*sin(beta(i)) / (w(i) - length2(i)*cos(beta(i)));
            end
        end

        % Determine slope of line from right vertex to midpoint of line from left vertex to peak.
        slope2 = ones(size(Target_Table, 1), 1) .* INT_MAX;

        for i=1:size(Target_Table, 1)
            if abs(w(i) - length1(i)*cos(alpha(i))) > 0.0
                slope2(i) = -length1(i)*sin(alpha(i)) / (w(i) - length1(i)*cos(alpha(i)));
            end
        end

        % Calculate centroid position.
        centroid_x = -(m.*slope2 + n.*slope1) ./ (slope1 - slope2);
        centroid_y = slope1.*(centroid_x + n);

        % Test if the point is under the left side of the peak.
        is_under_left = false(size(Target_Table, 1), 1);

        for i=1:size(Target_Table, 1)
            if n(i) >= 0
                is_under_left(i) = (h(i) + (h(i)/n(i)) * (xrotate(i) + centroid_x(i))) >= (yrotate(i) + centroid_y(i));
            else
                is_under_left(i) = (h(i) + (h(i)/n(i)) * (xrotate(i) + centroid_x(i))) <= (yrotate(i) + centroid_y(i));
            end
        end
        
        % Test if the point is under the right side of the peak.
        is_under_right = false(size(Target_Table, 1), 1);

        for i=1:size(Target_Table, 1)
            if m(i) >= 0
                is_under_right(i) = (h(i) - (h(i)/m(i)) * (xrotate(i) + centroid_x(i))) >= (yrotate(i) + centroid_y(i));
            else
                is_under_right(i) = (h(i) - (h(i)/m(i)) * (xrotate(i) + centroid_x(i))) <= (yrotate(i) + centroid_y(i));
            end
        end
        
        intarget(:,target) = is_under_right & ...            %under right side of peak
                             is_under_left & ...             %under left side of peak
                             (yrotate + centroid_y) >= 0.0;  %above base
    end
end

== matlab function KINARM_HandFeedbackInTarget/Embedded MATLAB WhichHand ==
  settings: fimath=|
      | fimath(...
      | 'RoundMode', 'floor',...
      | 'OverflowMode', 'wrap',...
      | 'ProductMode', 'KeepLSB', 'ProductWordLength', 32,...
      | 'SumMode', 'KeepLSB', 'SumWordLength', 32,...
      | 'CastBeforeSum', false)
  data: use_dominant_hand input double; dominant_hand input double; hand output double; cursor output double
function [hand, cursor] = WhichHand(use_dominant_hand, dominant_hand)

if use_dominant_hand==1				%use the dominant hand
	hand=dominant_hand;		
	cursor = 1;
else
	hand=3-dominant_hand;			%use the non-dominant hand. i.e. if dominant_hand=2, hand=1 and vice-versa
	cursor = 2;
end
